simulink model "fir_dbl_col_test"  (Simulink 7.2)
settings: Solver=FixedStepDiscrete  StartTime=0.0  StopTime=100  RelTol=1e-3
libraries: xbsIndex_r4 x31, casper_library_downconverter x4
settings Model: Creator=User  LastModifiedBy=root
settings OptimizationCC: InitFltsAndDblsToZero=on

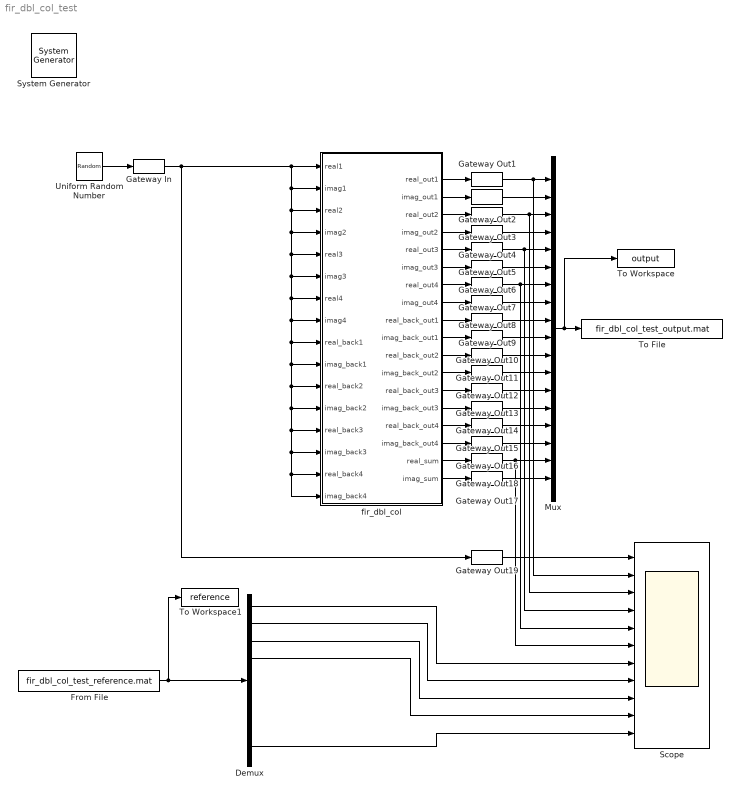
== system fir_dbl_col_test ==
  " System Generator" : xbsIndex_r4/ System Generator  Tag=genX  SystemSampleTime=-1  xilinxfamily=Virtex4  part=xc4vsx35  speed=-10  package=ff668  synthesis_tool=XST  clock_wrapper=Clock Enables  directory=./netlist  testbench=off  simulink_period=1  sysclk_period=100  dcm_input_clock_period=100  incr_netlist=off  trim_vbits=Everywhere in SubSystem  dbl_ovrd=According to Block Masks  core_generation=According to Block Masks  run_coregen=off  deprecated_control=off  eval_field=0  block_type=sysgen
      settings: block_version=10.1.1
  Demux : Demux  Outputs=18
  From File : FromFile  FileName=fir_dbl_col_test_reference.mat  SampleTime=1
  Gateway In : xbsIndex_r4/Gateway In  arith_type="Signed  (2's comp)"  n_bits=16  bin_pt=15  quantization="Round  (unbiased: +/- Inf)"  overflow=Saturate  period=1  dbl_ovrd=off  timing_constraint=None  locs_specified=off  LOCs={}  hdl_port=on  block_type=gatewayin
      settings: infoedit="Gateway in block.  Converts inputs of type Simulink integer, double and fixed point to  Xilinx fixed point type.<P><P>Hardware notes:  In hardware these blocks become top level input ports."  block_version=10.1.1
  Gateway Out{1..19} (19 alike) : xbsIndex_r4/Gateway Out  hdl_port=on  timing_constraint=None  locs_specified=off  LOCs={}  block_type=gatewayout
      settings: infoedit="Gateway out block.  Converts Xilinx fixed point inputs into ouputs of type Simulink integer, double, or fixed point.<P><P>Hardware notes:  In hardware these blocks become top level output ports or are discarded, depending on how they are configured."  block_version=10.1.1
  Mux : Mux  Inputs=18
  Scope : Scope  NumInputPorts=11
      settings: YMin=-5~-5~-5~-5~-5~-5~-5~-5~-5~-5~-5  YMax=5~5~5~5~5~5~5~5~5~5~5
  To File : ToFile  Filename=fir_dbl_col_test_output.mat  MatrixName=output
  To Workspace : ToWorkspace  VariableName=output  SampleTime=-1  SaveFormat=Array
  To Workspace1 : ToWorkspace  VariableName=reference  SampleTime=-1  SaveFormat=Array
  Uniform Random Number : UniformRandomNumber  SampleTime=1
  fir_dbl_col : Subsystem  AncestorBlock=casper_library_downconverter/fir_dbl_col  mask(fir_dbl_col){n_inputs=4, coeff=getfield( getfield( get_param( gcb,'UserData' ), 'parameters'),'coeff'), add_latency=2, mult_latency=2, coeff_bit_width=18, coeff_bin_pt=17, first_stage_hdl=on, adder_imp=DSP48}
      mask prompts: n_inputs "Inputs"; coeff "Coefficients"; add_latency "Add latency"; mult_latency "Mult Latency"; coeff_bit_width "Coefficient bit width"; coeff_bin_pt "Coefficient binary point"; first_stage_hdl "Implement first stage of adder trees on output as behavioural HDL"; adder_imp "Adder implementation"
      mask init:
      | fir_dbl_col_init(gcb, ...
      |     'n_inputs', n_inputs, ...
      |     'coeff', coeff, ...
      |     'mult_latency', mult_latency, ...
      |     'add_latency', add_latency, ...
      |     'coeff_bit_width', coeff_bit_width, ...
      |     'coeff_bin_pt', coeff_bin_pt,  ...
      |     'first_stage_hdl', first_stage_hdl, ...
      |     'adder_imp', adder_imp);
      mask Help: eval('xlWeb(''http://casper.berkeley.edu/wiki/Fir_dbl_col'')')
      mask StyleString: edit,edit,edit,edit,edit,edit,checkbox,popup(Behavioral|Fabric|DSP48)
  wires:
  Uniform Random Number/1 -> Gateway In/1
  Gateway In/1 -> fir_dbl_col/16(imag_back4), fir_dbl_col/15(real_back4), fir_dbl_col/14(imag_back3), fir_dbl_col/13(real_back3), fir_dbl_col/12(imag_back2), fir_dbl_col/11(real_back2), fir_dbl_col/10(imag_back1), fir_dbl_col/9(real_back1), fir_dbl_col/8(imag4), fir_dbl_col/7(real4), fir_dbl_col/6(imag3), fir_dbl_col/5(real3), fir_dbl_col/4(imag2), fir_dbl_col/3(real2), fir_dbl_col/2(imag1), fir_dbl_col/1(real1), Gateway Out19/1
  fir_dbl_col/1(real_out1) -> Gateway Out1/1
  fir_dbl_col/2(imag_out1) -> Gateway Out2/1
  fir_dbl_col/3(real_out2) -> Gateway Out3/1
  fir_dbl_col/4(imag_out2) -> Gateway Out4/1
  fir_dbl_col/5(real_out3) -> Gateway Out5/1
  fir_dbl_col/6(imag_out3) -> Gateway Out6/1
  fir_dbl_col/7(real_out4) -> Gateway Out7/1
  fir_dbl_col/8(imag_out4) -> Gateway Out8/1
  fir_dbl_col/9(real_back_out1) -> Gateway Out9/1
  fir_dbl_col/10(imag_back_out1) -> Gateway Out10/1
  fir_dbl_col/11(real_back_out2) -> Gateway Out11/1
  fir_dbl_col/12(imag_back_out2) -> Gateway Out12/1
  fir_dbl_col/13(real_back_out3) -> Gateway Out13/1
  fir_dbl_col/14(imag_back_out3) -> Gateway Out14/1
  fir_dbl_col/15(real_back_out4) -> Gateway Out15/1
  fir_dbl_col/16(imag_back_out4) -> Gateway Out16/1
  fir_dbl_col/17(real_sum) -> Gateway Out18/1
  fir_dbl_col/18(imag_sum) -> Gateway Out17/1
  Mux/1 -> To File/1, To Workspace/1
  Gateway Out1/1 -> Mux/1, Scope/2
  Gateway Out2/1 -> Mux/2
  Gateway Out3/1 -> Mux/3, Scope/3
  Gateway Out4/1 -> Mux/4
  Gateway Out5/1 -> Mux/5, Scope/4
  Gateway Out6/1 -> Mux/6
  Gateway Out7/1 -> Mux/7, Scope/5
  Gateway Out8/1 -> Mux/8
  Gateway Out9/1 -> Mux/9
  Gateway Out10/1 -> Mux/10
  Gateway Out11/1 -> Mux/11
  Gateway Out12/1 -> Mux/12
  Gateway Out13/1 -> Mux/13
  Gateway Out14/1 -> Mux/14
  Gateway Out15/1 -> Mux/15
  Gateway Out16/1 -> Mux/16
  Gateway Out17/1 -> Mux/18
  Gateway Out18/1 -> Mux/17, Scope/6
  Gateway Out19/1 -> Scope/1
  From File/1 -> Demux/1, To Workspace1/1
  Demux/1 -> Scope/7
  Demux/3 -> Scope/8
  Demux/5 -> Scope/9
  Demux/7 -> Scope/10
  Demux/17 -> Scope/11

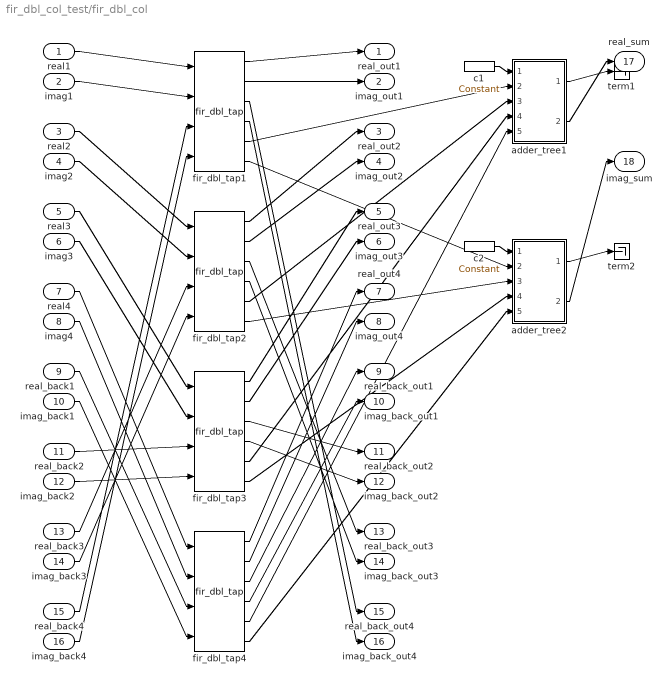
== system fir_dbl_col_test/fir_dbl_col ==
  real1 : Inport
  imag1 : Inport  Port=2
  real2 : Inport  Port=3
  imag2 : Inport  Port=4
  real3 : Inport  Port=5
  imag3 : Inport  Port=6
  real4 : Inport  Port=7
  imag4 : Inport  Port=8
  real_back1 : Inport  Port=9
  imag_back1 : Inport  Port=10
  real_back2 : Inport  Port=11
  imag_back2 : Inport  Port=12
  real_back3 : Inport  Port=13
  imag_back3 : Inport  Port=14
  real_back4 : Inport  Port=15
  imag_back4 : Inport  Port=16
  adder_tree1 : Subsystem  AncestorBlock=casper_library_misc/adder_tree  mask(adder_tree){n_inputs=4, latency=2, adder_imp=DSP48, first_stage_hdl=on}
      mask prompts: n_inputs "Number of Inputs"; latency "Add Latency"; adder_imp "Adder implementation"; first_stage_hdl "Use behavioural HDL for first stage of adders"
      mask help:
      | Sums all inputs using a tree of adds and delays.
      |
      | Number of inputs: The number of inputs to the block to be summed
      | Add latency: The number of clock cycles to perform one addition (affects timing)..
      | Adder implementation: choice of fabric or DSP48E core, or behavioral HDL
      | Use behavioural HDL for first stage of adders: Causes the first stage of adders to be absorbed into DSP blocks if multipliers precede them (Virtex 5). Overrides Adder implementation
      mask init:
      | adder_tree_init(gcb, ...
      |     'n_inputs', n_inputs, ...
      |     'latency', latency, ...
      |     'adder_imp', adder_imp, ...
      |     'first_stage_hdl', first_stage_hdl);
      settings: AttributesFormatString=latency 4
      mask Help: eval('xlWeb(''http://casper.berkeley.edu/wiki/Adder_tree'')')
      mask StyleString: edit,edit,popup(Behavioral|Fabric|DSP48),checkbox
  adder_tree2 : Subsystem  AncestorBlock=casper_library_misc/adder_tree  mask(adder_tree){n_inputs=4, latency=2, adder_imp=DSP48, first_stage_hdl=on}
      mask prompts: n_inputs "Number of Inputs"; latency "Add Latency"; adder_imp "Adder implementation"; first_stage_hdl "Use behavioural HDL for first stage of adders"
      mask help:
      | Sums all inputs using a tree of adds and delays.
      |
      | Number of inputs: The number of inputs to the block to be summed
      | Add latency: The number of clock cycles to perform one addition (affects timing)..
      | Adder implementation: choice of fabric or DSP48E core, or behavioral HDL
      | Use behavioural HDL for first stage of adders: Causes the first stage of adders to be absorbed into DSP blocks if multipliers precede them (Virtex 5). Overrides Adder implementation
      mask init:
      | adder_tree_init(gcb, ...
      |     'n_inputs', n_inputs, ...
      |     'latency', latency, ...
      |     'adder_imp', adder_imp, ...
      |     'first_stage_hdl', first_stage_hdl);
      settings: AttributesFormatString=latency 4
      mask Help: eval('xlWeb(''http://casper.berkeley.edu/wiki/Adder_tree'')')
      mask StyleString: edit,edit,popup(Behavioral|Fabric|DSP48),checkbox
  c1 : xbsIndex_r4/Constant  arith_type=Signed (2's comp)  const=1  n_bits=16  bin_pt=14  explicit_period=on  period=1  equ=P=C  opselect=C  inp2=PCIN>>17  opr=+  inp1=P  carry=CIN  dbl_ovrd=off  block_type=constant
      settings: block_version=11.4
  c2 : xbsIndex_r4/Constant  arith_type=Signed (2's comp)  const=1  n_bits=16  bin_pt=14  explicit_period=on  period=1  equ=P=C  opselect=C  inp2=PCIN>>17  opr=+  inp1=P  carry=CIN  dbl_ovrd=off  block_type=constant
      settings: block_version=11.4
  fir_dbl_tap1 : casper_library_downconverter/fir_dbl_tap  SystemSampleTime=-1  factor=0.1  add_latency=2  mult_latency=2  coeff_bit_width=18  coeff_bin_pt=17
  fir_dbl_tap2 : casper_library_downconverter/fir_dbl_tap  SystemSampleTime=-1  factor=0.2  add_latency=2  mult_latency=2  coeff_bit_width=18  coeff_bin_pt=17
  fir_dbl_tap3 : casper_library_downconverter/fir_dbl_tap  SystemSampleTime=-1  factor=0.3  add_latency=2  mult_latency=2  coeff_bit_width=18  coeff_bin_pt=17
  fir_dbl_tap4 : casper_library_downconverter/fir_dbl_tap  SystemSampleTime=-1  factor=0.4  add_latency=2  mult_latency=2  coeff_bit_width=18  coeff_bin_pt=17
  term1 : Terminator
  term2 : Terminator
  real_out1 : Outport
  imag_out1 : Outport  Port=2
  real_out2 : Outport  Port=3
  imag_out2 : Outport  Port=4
  real_out3 : Outport  Port=5
  imag_out3 : Outport  Port=6
  real_out4 : Outport  Port=7
  imag_out4 : Outport  Port=8
  real_back_out1 : Outport  Port=9
  imag_back_out1 : Outport  Port=10
  real_back_out2 : Outport  Port=11
  imag_back_out2 : Outport  Port=12
  real_back_out3 : Outport  Port=13
  imag_back_out3 : Outport  Port=14
  real_back_out4 : Outport  Port=15
  imag_back_out4 : Outport  Port=16
  real_sum : Outport  Port=17
  imag_sum : Outport  Port=18
  wires:
  adder_tree1/1(sync_out) -> term1/1
  adder_tree2/1(sync_out) -> term2/1
  c1/1 -> adder_tree1/1(sync)
  c2/1 -> adder_tree2/1(sync)
  adder_tree1/2(dout) -> real_sum/1
  adder_tree2/2(dout) -> imag_sum/1
  real1/1 -> fir_dbl_tap1/1
  imag1/1 -> fir_dbl_tap1/2
  real_back4/1 -> fir_dbl_tap1/3
  imag_back4/1 -> fir_dbl_tap1/4
  fir_dbl_tap1/1 -> real_out1/1
  fir_dbl_tap1/2 -> imag_out1/1
  fir_dbl_tap1/3 -> real_back_out4/1
  fir_dbl_tap1/4 -> imag_back_out4/1
  fir_dbl_tap1/5 -> adder_tree1/2(din1)
  fir_dbl_tap1/6 -> adder_tree2/2(din1)
  real2/1 -> fir_dbl_tap2/1
  imag2/1 -> fir_dbl_tap2/2
  real_back3/1 -> fir_dbl_tap2/3
  imag_back3/1 -> fir_dbl_tap2/4
  fir_dbl_tap2/1 -> real_out2/1
  fir_dbl_tap2/2 -> imag_out2/1
  fir_dbl_tap2/3 -> real_back_out3/1
  fir_dbl_tap2/4 -> imag_back_out3/1
  fir_dbl_tap2/5 -> adder_tree1/3(din2)
  fir_dbl_tap2/6 -> adder_tree2/3(din2)
  real3/1 -> fir_dbl_tap3/1
  imag3/1 -> fir_dbl_tap3/2
  real_back2/1 -> fir_dbl_tap3/3
  imag_back2/1 -> fir_dbl_tap3/4
  fir_dbl_tap3/1 -> real_out3/1
  fir_dbl_tap3/2 -> imag_out3/1
  fir_dbl_tap3/3 -> real_back_out2/1
  fir_dbl_tap3/4 -> imag_back_out2/1
  fir_dbl_tap3/5 -> adder_tree1/4(din3)
  fir_dbl_tap3/6 -> adder_tree2/4(din3)
  real4/1 -> fir_dbl_tap4/1
  imag4/1 -> fir_dbl_tap4/2
  real_back1/1 -> fir_dbl_tap4/3
  imag_back1/1 -> fir_dbl_tap4/4
  fir_dbl_tap4/1 -> real_out4/1
  fir_dbl_tap4/2 -> imag_out4/1
  fir_dbl_tap4/3 -> real_back_out1/1
  fir_dbl_tap4/4 -> imag_back_out1/1
  fir_dbl_tap4/5 -> adder_tree1/5(din4)
  fir_dbl_tap4/6 -> adder_tree2/5(din4)

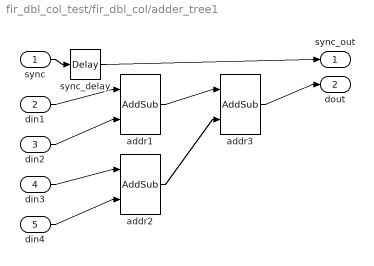
== system fir_dbl_col_test/fir_dbl_col/adder_tree1 ==
  sync : Inport
  din1 : Inport  Port=2
  din2 : Inport  Port=3
  din3 : Inport  Port=4
  din4 : Inport  Port=5
  addr1 : xbsIndex_r4/AddSub  mode=Addition  use_carryin=off  use_carryout=off  en=off  latency=2  precision=Full  arith_type=Unsigned  n_bits=16  bin_pt=14  quantization=Truncate  overflow=Wrap  dbl_ovrd=off  use_behavioral_HDL=on  hw_selection=DSP48  pipelined=on  use_rpm=on  block_type=addsub
  addr2 : xbsIndex_r4/AddSub  mode=Addition  use_carryin=off  use_carryout=off  en=off  latency=2  precision=Full  arith_type=Unsigned  n_bits=16  bin_pt=14  quantization=Truncate  overflow=Wrap  dbl_ovrd=off  use_behavioral_HDL=on  hw_selection=DSP48  pipelined=on  use_rpm=on  block_type=addsub
  addr3 : xbsIndex_r4/AddSub  mode=Addition  use_carryin=off  use_carryout=off  en=off  latency=2  precision=Full  arith_type=Unsigned  n_bits=16  bin_pt=14  quantization=Truncate  overflow=Wrap  dbl_ovrd=off  use_behavioral_HDL=off  hw_selection=DSP48  pipelined=on  use_rpm=on  block_type=addsub
  sync_delay : xbsIndex_r4/Delay  en=off  latency=4  dbl_ovrd=off  reg_retiming=on  block_type=delay
      settings: block_version=11.4
  sync_out : Outport
  dout : Outport  Port=2
  wires:
  sync/1 -> sync_delay/1
  sync_delay/1 -> sync_out/1
  din1/1 -> addr1/1
  din2/1 -> addr1/2
  din3/1 -> addr2/1
  din4/1 -> addr2/2
  addr1/1 -> addr3/1
  addr2/1 -> addr3/2
  addr3/1 -> dout/1

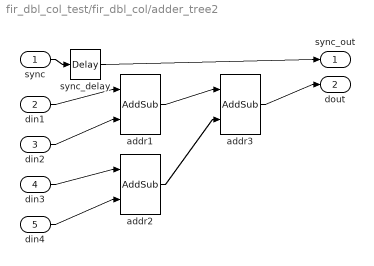
== system fir_dbl_col_test/fir_dbl_col/adder_tree2 ==
  sync : Inport
  din1 : Inport  Port=2
  din2 : Inport  Port=3
  din3 : Inport  Port=4
  din4 : Inport  Port=5
  addr1 : xbsIndex_r4/AddSub  mode=Addition  use_carryin=off  use_carryout=off  en=off  latency=2  precision=Full  arith_type=Unsigned  n_bits=16  bin_pt=14  quantization=Truncate  overflow=Wrap  dbl_ovrd=off  use_behavioral_HDL=on  hw_selection=DSP48  pipelined=on  use_rpm=on  block_type=addsub
  addr2 : xbsIndex_r4/AddSub  mode=Addition  use_carryin=off  use_carryout=off  en=off  latency=2  precision=Full  arith_type=Unsigned  n_bits=16  bin_pt=14  quantization=Truncate  overflow=Wrap  dbl_ovrd=off  use_behavioral_HDL=on  hw_selection=DSP48  pipelined=on  use_rpm=on  block_type=addsub
  addr3 : xbsIndex_r4/AddSub  mode=Addition  use_carryin=off  use_carryout=off  en=off  latency=2  precision=Full  arith_type=Unsigned  n_bits=16  bin_pt=14  quantization=Truncate  overflow=Wrap  dbl_ovrd=off  use_behavioral_HDL=off  hw_selection=DSP48  pipelined=on  use_rpm=on  block_type=addsub
  sync_delay : xbsIndex_r4/Delay  en=off  latency=4  dbl_ovrd=off  reg_retiming=on  block_type=delay
      settings: block_version=11.4
  sync_out : Outport
  dout : Outport  Port=2
  wires:
  sync/1 -> sync_delay/1
  sync_delay/1 -> sync_out/1
  din1/1 -> addr1/1
  din2/1 -> addr1/2
  din3/1 -> addr2/1
  din4/1 -> addr2/2
  addr1/1 -> addr3/1
  addr2/1 -> addr3/2
  addr3/1 -> dout/1
